simulink model "Cuves_PROFIBUS_Stateflow"  (R2024a)
settings: Solver=FixedStepDiscrete  StartTime=0.0  StopTime=65  FixedStep=0.01  RelTol=1e-3
model workspace (MAT data in the model file):
  scenarioData.time = [0; 1; 1.3; 65]
  scenarioData.signals.values = [0  0  0  0  0  0; 1  0  0  0  0  0; 0  0  0  0  0  0; 0  0  0  0  0  0]
  scenarioData.signals.dimensions = 6
settings Model: Creator=DIAW  LastModifiedBy=DIAW
settings OptimizationCC: BlockReduction=off  OptimizeBlockIOStorage=off

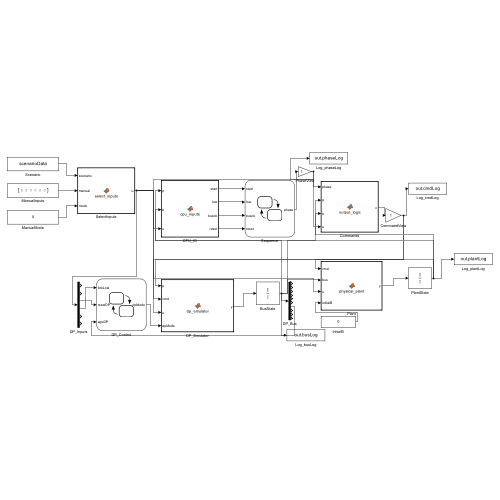
[thumbnail: Simulink's stored preview of the top-level diagram]
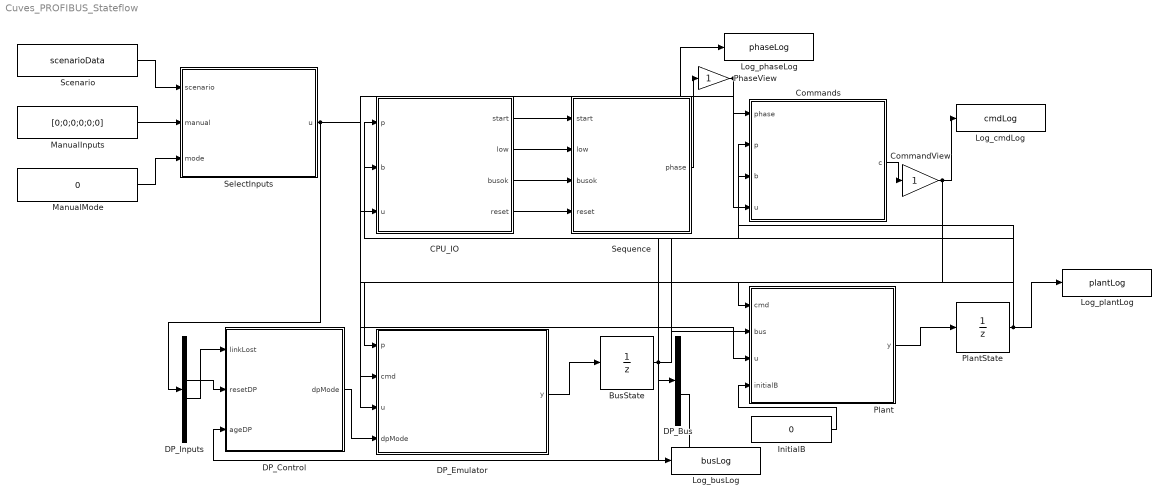
== system Cuves_PROFIBUS_Stateflow ==
  BusState : UnitDelay  InitialCondition=zeros(10,1)  SampleTime=0.01  HasFrameUpgradeWarning=on
  CPU_IO : MATLAB Function  TreatAsAtomicUnit=on
  CommandView : Gain
  Commands : MATLAB Function  TreatAsAtomicUnit=on
  DP_Bus : Demux  Outputs=10
  DP_Control : Stateflow chart  TreatAsAtomicUnit=on
  DP_Emulator : MATLAB Function  TreatAsAtomicUnit=on
  DP_Inputs : Demux  Outputs=6
  InitialB : Constant  Value=0  SampleTime=0.01
  Log_busLog : ToWorkspace  VariableName=busLog  SaveFormat=Structure With Time  SampleTime=-1
  Log_cmdLog : ToWorkspace  VariableName=cmdLog  SaveFormat=Structure With Time  SampleTime=-1
  Log_phaseLog : ToWorkspace  VariableName=phaseLog  SaveFormat=Structure With Time  SampleTime=-1
  Log_plantLog : ToWorkspace  VariableName=plantLog  SaveFormat=Structure With Time  SampleTime=-1
  ManualInputs : Constant  Value=[0;0;0;0;0;0]  SampleTime=0.01
  ManualMode : Constant  Value=0  SampleTime=0.01
  PhaseView : Gain
  Plant : MATLAB Function  TreatAsAtomicUnit=on
  PlantState : UnitDelay  InitialCondition=[0;0;0;1;0;0;0;0]  SampleTime=0.01  HasFrameUpgradeWarning=on
  Scenario : FromWorkspace  VariableName=scenarioData  SampleTime=0.01  Interpolate=off  OutputAfterFinalValue=Holding final value
  SelectInputs : MATLAB Function  TreatAsAtomicUnit=on
  Sequence : Stateflow chart  TreatAsAtomicUnit=on
  wires:
  Scenario/1 -> SelectInputs/1(scenario)
  ManualInputs/1 -> SelectInputs/2(manual)
  ManualMode/1 -> SelectInputs/3(mode)
  PlantState/1 -> CPU_IO/1(p), Commands/2(p), DP_Emulator/1(p), Log_plantLog/1
  BusState/1 -> CPU_IO/2(b), Commands/3(b), DP_Bus/1, Plant/2(bus), Log_busLog/1
  SelectInputs/1(u) -> CPU_IO/3(u), Commands/4(u), DP_Inputs/1, DP_Emulator/3(u), Plant/3(u)
  CPU_IO/1(start) -> Sequence/1(start)
  CPU_IO/2(low) -> Sequence/2(low)
  CPU_IO/3(busok) -> Sequence/3(busok)
  CPU_IO/4(reset) -> Sequence/4(reset)
  Sequence/1(phase) -> PhaseView/1
  PhaseView/1 -> Commands/1(phase), Log_phaseLog/1
  DP_Inputs/4 -> DP_Control/1(linkLost)
  DP_Inputs/3 -> DP_Control/2(resetDP)
  DP_Bus/7 -> DP_Control/3(ageDP)
  Commands/1(c) -> CommandView/1
  CommandView/1 -> DP_Emulator/2(cmd), Plant/1(cmd), Log_cmdLog/1
  DP_Control/1(dpMode) -> DP_Emulator/4(dpMode)
  DP_Emulator/1(y) -> BusState/1
  InitialB/1 -> Plant/4(initialB)
  Plant/1(y) -> PlantState/1

== matlab function Cuves_PROFIBUS_Stateflow/CPU_IO ==
  settings: updateMethod=DISCRETE  sampleTime=0.01
  data: p input; b input; u input; start output; low output; busok output; reset output
function [start,low,busok,reset] = cpu_inputs(p,b,u)
%#codegen
persistent old1 old2
if isempty(old1), old1=false; old2=false; end
s1=u(1)>0.5; s2=b(2)>0.5;
start=double((s1 && ~old1) || (s2 && ~old2));
old1=s1; old2=s2;
low=p(4); busok=b(5); reset=u(3);
if reset>0.5, start=0; end
end

== matlab function Cuves_PROFIBUS_Stateflow/SelectInputs ==
  settings: updateMethod=DISCRETE  sampleTime=0.01
  data: scenario input; u output; manual input; mode input
function u = select_inputs(scenario,manual,mode)
%#codegen
u=zeros(6,1);
for k=1:6
    if mode>0.5, u(k)=manual(k); else, u(k)=scenario(k); end
end
end

== matlab function Cuves_PROFIBUS_Stateflow/Commands ==
  settings: updateMethod=DISCRETE  sampleTime=0.01
  data: phase input; p input; b input; u input; c output
function c = output_logic(phase,p,b,u)
%#codegen
c=zeros(5,1);
if b(5)>0.5 && u(3)<0.5
    c(1)=double(phase==1); c(2)=double(phase==2);
    c(3)=double(phase==3); c(5)=double(phase==4);
    c(4)=double(phase==4 && b(3)>0.5 && b(4)<0.5 && p(4)<0.5);
end
end

== matlab function Cuves_PROFIBUS_Stateflow/DP_Emulator ==
  settings: updateMethod=DISCRETE  sampleTime=0.01
  data: p input; cmd input; u input; y output; dpMode input
function y = dp_emulator(p,cmd,u,dpMode)
%#codegen
% EMULATION FONCTIONNELLE DP : pas une pile FDL ni une interface RS-485.
% Donnees 16 DI/16 DQ ET200M. Deuxieme octet toujours nul et reserve.
% y: VA03, DCY2, FDCO, NH_B, ok, cycles, age_s, tx0, rx0, etat_DP
persistent tick age cycles lastMode remote rx haveData
if isempty(tick)
    tick=0; age=0; cycles=0; lastMode=-1; remote=0; rx=uint8(0); haveData=false;
end
if u(3)>0.5
    tick=0; age=0; cycles=0; lastMode=-1; remote=0; rx=uint8(0); haveData=false;
end
% Stateflow decide de l'etat du maitre. Ce bloc traite les octets en ECHANGE.
if dpMode~=lastMode
    age=0; haveData=false; remote=0; lastMode=dpMode;
end
tick=tick+1; age=age+0.01;
tx=uint8(0); tx=bitset(tx,1,cmd(5)>0.5);
if dpMode==3 && mod(tick,2)==0 && u(4)<0.5
    % Encode et decode reellement les octets de donnees utilisateur.
    inputBytes=zeros(2,1,'uint8'); outputBytes=zeros(2,1,'uint8');
    outputBytes(1)=tx;
    inputBytes(1)=bitset(inputBytes(1),1,u(2)>0.5);
    inputBytes(1)=bitset(inputBytes(1),2,p(6)>0.5);
    inputBytes(1)=bitset(inputBytes(1),3,p(5)>0.5);
    remote=double(bitget(outputBytes(1),1));
    rx=inputBytes(1); age=0; cycles=cycles+1; haveData=true;
end
ok=double(dpMode==3 && age<0.10 && haveData && u(4)<0.5);
if age>=0.10 || u(4)>0.5
    remote=0; ok=0; haveData=false; % valeur de repli choisie pour la simulation
end
y=[remote;double(bitget(rx,1));double(bitget(rx,2));...
   double(bitget(rx,3));ok;cycles;age;double(tx);double(rx);dpMode];
end

== matlab function Cuves_PROFIBUS_Stateflow/Plant ==
  settings: updateMethod=DISCRETE  sampleTime=0.01
  data: cmd input; bus input; u input; y output; initialB input
function y = physical_plant(cmd,bus,u,initialB)
%#codegen
% Volumes L; discretisation 10 ms. Parametres pedagogiques, non identifies.
persistent a b pos spillA spillB
if isempty(a)
    a=0; b=initialB; pos=0; spillA=0; spillB=0;
end
if u(3)>0.5
    a=0; b=initialB; pos=0; spillA=0; spillB=0;
else
    if u(5)>0.5
        target=0; % vanne bloquee fermee
    else
        target=bus(1); % COMMANDE DEPORTEE, pas cmd(5) directement
    end
    pos=pos+min(0.01/0.4,1)*(target-pos);
    qin=2*cmd(1)+3*cmd(2);
    qtransfer=min(4*cmd(4)*pos,a/0.01);
    qdrain=min(3*double(u(6)>0.5),b/0.01);
    rawA=a+0.01*(qin-qtransfer);
    rawB=b+0.01*(qtransfer-qdrain);
    spillA=spillA+max(0,rawA-100);
    spillB=spillB+max(0,rawB-100);
    a=min(100,max(0,rawA)); b=min(100,max(0,rawB));
end
y=[a;b;pos;double(a<=2);double(b>=90);double(pos>=0.95);spillA;spillB];
end

== stateflow chart Cuves_PROFIBUS_Stateflow/Sequence ==
  settings: updateMethod=DISCRETE  sampleTime=0.01
  state CYCLE_CPU
    state REMPLISSAGE_P1
      entry:
      phase = 1;
      during:
      phase = 1;
    state REMPLISSAGE_P2
      entry:
      phase = 2;
      during:
      phase = 2;
    state AGITATION
      entry:
      phase = 3;
      during:
      phase = 3;
    state TRANSFERT
      entry:
      phase = 4;
      during:
      phase = 4;
    (default) -> REMPLISSAGE_P1
    REMPLISSAGE_P1 -> REMPLISSAGE_P2 : after(10,sec)
    REMPLISSAGE_P2 -> AGITATION : after(5,sec)
    AGITATION -> TRANSFERT : after(15,sec)
  state ATTENTE
    entry:
    phase = 0;
    during:
    phase = 0;
  state DEFAUT_BUS
    entry:
    phase = 9;
    during:
    phase = 9;
  CYCLE_CPU -> ATTENTE [order 2] : [reset > 0.5]
  (default) -> ATTENTE
  ATTENTE -> CYCLE_CPU : [start > 0.5 && low > 0.5 && busok > 0.5 && reset < 0.5]
  CYCLE_CPU -> ATTENTE [order 3] : [phase == 4 && low > 0.5]
  DEFAUT_BUS -> ATTENTE : [reset > 0.5 && busok > 0.5]
  CYCLE_CPU -> DEFAUT_BUS [order 1] : [busok < 0.5]
  data: start input double; low input double; busok input double; reset input double; phase output double

== stateflow chart Cuves_PROFIBUS_Stateflow/DP_Control ==
  settings: updateMethod=DISCRETE  sampleTime=0.01
  state SERVICE_DP
    state PARAMETRAGE
      entry:
      dpMode = 1;
      during:
      dpMode = 1;
    state CONFIGURATION
      entry:
      dpMode = 2;
      during:
      dpMode = 2;
    state ECHANGE
      entry:
      dpMode = 3;
      during:
      dpMode = 3;
    (default) -> PARAMETRAGE
    PARAMETRAGE -> CONFIGURATION : after(0.02,sec)
    CONFIGURATION -> ECHANGE : after(0.02,sec)
  state ATTENTE
    entry:
    dpMode = 0;
    during:
    dpMode = 0;
  state DEFAUT_LIAISON
    entry:
    dpMode = 4;
    during:
    dpMode = 4;
  SERVICE_DP -> ATTENTE [order 2] : [resetDP > 0.5]
  (default) -> ATTENTE
  ATTENTE -> SERVICE_DP [order 2] : after(0.02,sec)
  DEFAUT_LIAISON -> ATTENTE : [linkLost < 0.5]
  ATTENTE -> DEFAUT_LIAISON [order 1] : [linkLost > 0.5]
  SERVICE_DP -> DEFAUT_LIAISON [order 1] : [linkLost > 0.5 || (dpMode == 3 && ageDP >= 0.10)]
  data: linkLost input double; resetDP input double; ageDP input double; dpMode output double
